simulink model "RobotDelta_NMPC"  (R2025b)
settings: Solver=daessc  StartTime=0.0  StopTime=10  MaxStep=1e-2  RelTol=1e-3
PreLoadFcn:
  | if isempty(which('RobotDelta_Params')), run(fullfile(fileparts(get_param(bdroot,'FileName')),'..','tools','rd_addpath.m')); end; RobotDelta_Params;
InitFcn:
  | RobotDelta_Params; addpath(fullfile(rd_root(), 'work'));
undefined symbols (not defined in the file): G, Nmpc, RobotDelta_IK, RobotDelta_Traj, smiData, Traj, X, Y, Z
libraries: sm_lib x256, nesl_utility x13
(part 1 of 6)
settings Model: Creator=nguye  LastModifiedBy=nguye

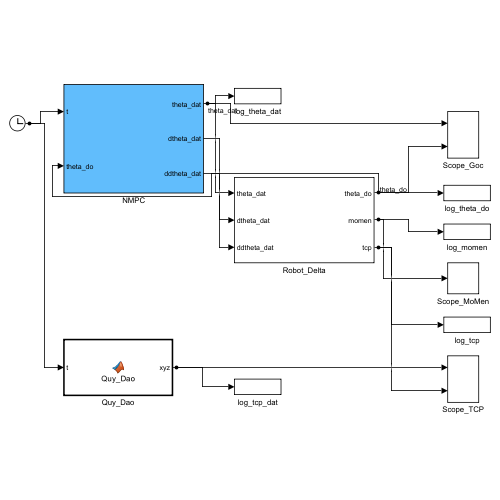
[thumbnail: Simulink's stored preview of the top-level diagram]
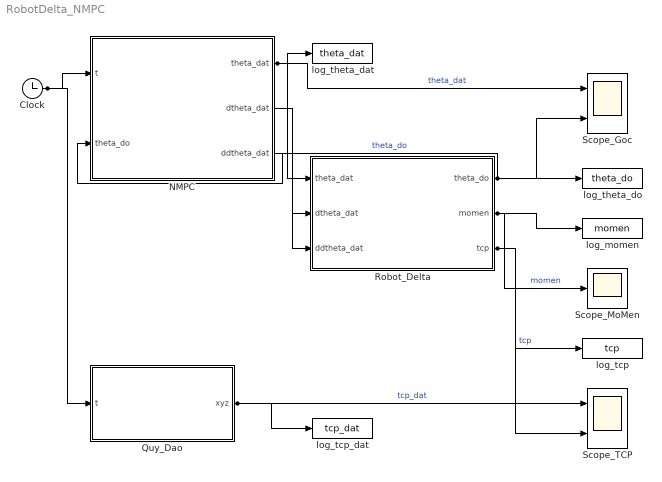
== system RobotDelta_NMPC ==
  Clock : Clock
  NMPC : Subsystem
  Quy_Dao : MATLAB Function  TreatAsAtomicUnit=on
  Robot_Delta : Subsystem
  Scope_Goc : Scope  NumInputPorts=2
  Scope_MoMen : Scope
  Scope_TCP : Scope  NumInputPorts=2
  log_momen : ToWorkspace  VariableName=momen  SaveFormat=Timeseries  SampleTime=-1
  log_tcp : ToWorkspace  VariableName=tcp  SaveFormat=Timeseries  SampleTime=-1
  log_tcp_dat : ToWorkspace  VariableName=tcp_dat  SaveFormat=Timeseries  SampleTime=-1
  log_theta_dat : ToWorkspace  VariableName=theta_dat  SaveFormat=Timeseries  SampleTime=-1
  log_theta_do : ToWorkspace  VariableName=theta_do  SaveFormat=Timeseries  SampleTime=-1
  wires:
  Robot_Delta/2(momen) -> Scope_MoMen/1, log_momen/1  "momen"
  Clock/1 -> Quy_Dao/1(t), NMPC/1(t)
  Quy_Dao/1(xyz) -> Scope_TCP/1, log_tcp_dat/1  "tcp_dat"
  Robot_Delta/1(theta_do) -> Scope_Goc/2, log_theta_do/1, NMPC/2(theta_do)  "theta_do"
  Robot_Delta/3(tcp) -> Scope_TCP/2, log_tcp/1  "tcp"
  NMPC/1(theta_dat) -> Scope_Goc/1, Robot_Delta/1(theta_dat), log_theta_dat/1  "theta_dat"
  NMPC/2(dtheta_dat) -> Robot_Delta/2(dtheta_dat)
  NMPC/3(ddtheta_dat) -> Robot_Delta/3(ddtheta_dat)

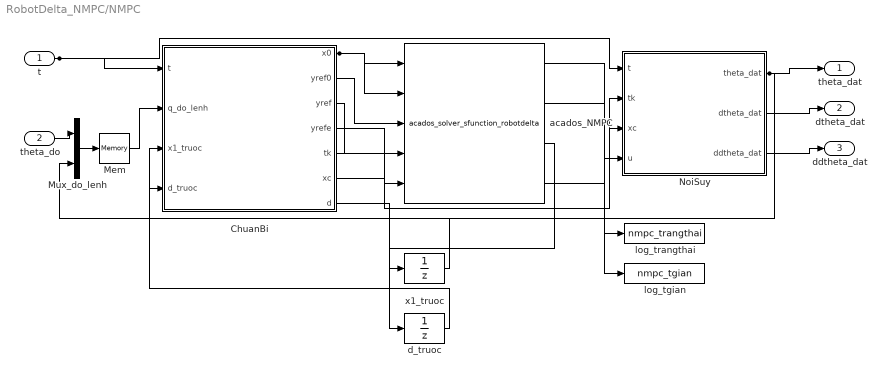
== system RobotDelta_NMPC/NMPC ==
  t : Inport
  theta_do : Inport  Port=2
  ChuanBi : MATLAB Function  TreatAsAtomicUnit=on
  Mem : Memory  InitialCondition=repmat(RobotDelta_IK(RobotDelta_Traj(0, Traj), G), 2, 1)
  Mux_do_lenh : Mux  Inputs=2
  NoiSuy : MATLAB Function  TreatAsAtomicUnit=on
  acados_NMPC : S-Function  FunctionName=acados_solver_sfunction_robotdelta  SFunctionDeploymentMode=off  EnableBusSupport=off
  d_truoc : UnitDelay  InitialCondition=zeros(3,1)  SampleTime=Nmpc.Ts  HasFrameUpgradeWarning=on
  log_tgian : ToWorkspace  VariableName=nmpc_tgian  SaveFormat=Timeseries  SampleTime=-1
  log_trangthai : ToWorkspace  VariableName=nmpc_trangthai  SaveFormat=Timeseries  SampleTime=-1
  x1_truoc : UnitDelay  InitialCondition=[RobotDelta_IK(RobotDelta_Traj(0, Traj), G)*pi/180; 0; 0; 0]  SampleTime=Nmpc.Ts  HasFrameUpgradeWarning=on
  theta_dat : Outport
  dtheta_dat : Outport  Port=2
  ddtheta_dat : Outport  Port=3
  wires:
  t/1 -> ChuanBi/1(t), NoiSuy/1(t)
  theta_do/1 -> Mux_do_lenh/1
  NoiSuy/1(theta_dat) -> Mux_do_lenh/2, theta_dat/1
  Mux_do_lenh/1 -> Mem/1
  Mem/1 -> ChuanBi/2(q_do_lenh)
  x1_truoc/1 -> ChuanBi/3(x1_truoc)
  d_truoc/1 -> ChuanBi/4(d_truoc)
  ChuanBi/7(d) -> d_truoc/1
  ChuanBi/1(x0) -> acados_NMPC/1, acados_NMPC/2
  ChuanBi/2(yref0) -> acados_NMPC/3
  ChuanBi/3(yref) -> acados_NMPC/4
  ChuanBi/4(yrefe) -> acados_NMPC/5
  acados_NMPC/3 -> x1_truoc/1
  ChuanBi/5(tk) -> NoiSuy/2(tk)
  ChuanBi/6(xc) -> NoiSuy/3(xc)
  acados_NMPC/1 -> NoiSuy/4(u)
  acados_NMPC/2 -> log_trangthai/1
  acados_NMPC/4 -> log_tgian/1
  NoiSuy/2(dtheta_dat) -> dtheta_dat/1
  NoiSuy/3(ddtheta_dat) -> ddtheta_dat/1

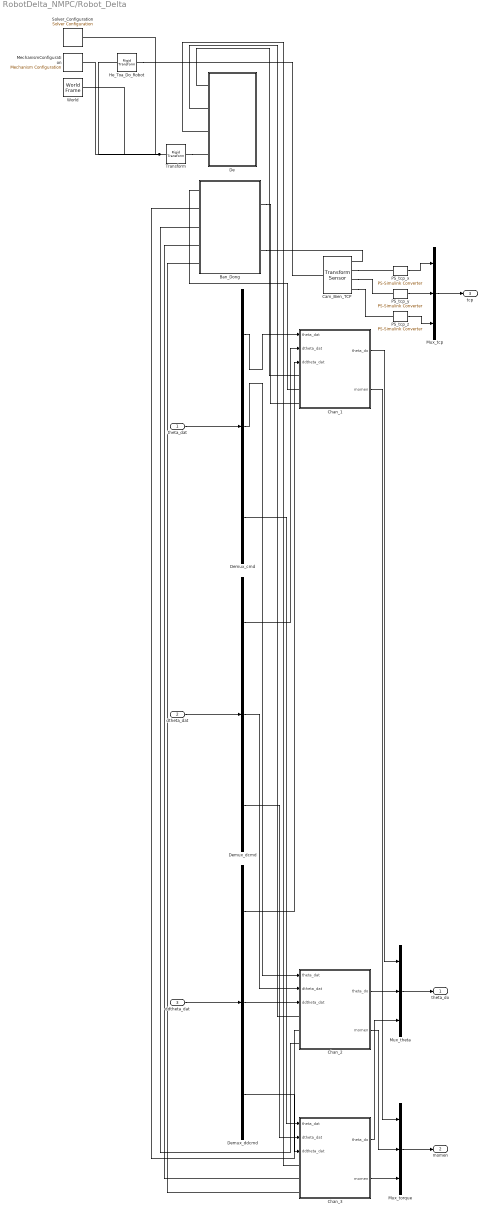
== system RobotDelta_NMPC/Robot_Delta ==
  theta_dat : Inport
  dtheta_dat : Inport  Port=2
  ddtheta_dat : Inport  Port=3
  Ban_Dong : Subsystem
  Cam_Bien_TCP : sm_lib/Frames and Transforms/Transform Sensor  MeasurementFrame=World  RotationSequence=XYX  SenseAngle=off  SenseAxis=off  SenseQ=off  SenseR=off  SenseRotationSequence=off  SenseOmegaX=off  SenseOmegaY=off  SenseOmegaZ=off  SenseOmega=off  SenseQDot=off  SenseRDot=off  SenseRotationSequenceDot=off  SenseAlphaX=off  SenseAlphaY=off  SenseAlphaZ=off  SenseAlpha=off  SenseQDDot=off  SenseRDDot=off  SenseX=on  SenseY=on  SenseZ=on  SenseXYZ=off  SenseRad=off  SenseAzim=off  SenseDist=off  SenseInc=off  SenseXDot=off  SenseYDot=off  SenseZDot=off  SenseXYZDot=off  SenseRadDot=off  SenseAzimDot=off  SenseDistDot=off  SenseIncDot=off  SenseXDDot=off  SenseYDDot=off  SenseZDDot=off  SenseXYZDDot=off  SenseRadDDot=off  SenseAzimDDot=off  SenseDistDDot=off  SenseIncDDot=off
  Chan_1 : Subsystem
  Chan_2 : Subsystem
  Chan_3 : Subsystem
  De : Subsystem
  Demux_cmd : Demux  Outputs=3
  Demux_dcmd : Demux  Outputs=3
  Demux_ddcmd : Demux  Outputs=3
  He_Toa_Do_Robot : sm_lib/Frames and Transforms/Rigid Transform  RotationMethod=None  FollAlignAxisA=+X  BaseAlignAxisA=+Y  FollAlignAxisB=+Y  BaseAlignAxisB=+Z  RotationStandardAxis=+Z  RotationAngle=0  RotationAngleUnits=deg  RotationArbitraryAxis=[0 0 1]  RotationSequenceAxes=FollowerAxes  RotationSequence=XYX  RotationSequenceAngles=[0 0 0]  RotationSequenceAnglesUnits=deg  RotationMatrix=[1 0 0;0 1 0;0 0 1]  Quaternion=[1 0 0 0]  TranslationMethod=Cartesian  TranslationCartesianOffset=G.origin  TranslationCartesianOffsetUnits=m  TranslationStandardAxis=+Z  TranslationStandardOffset=0  TranslationStandardOffsetUnits=m  TranslationROffset=0  TranslationROffsetUnits=m  TranslationThetaOffset=0  TranslationThetaOffsetUnits=deg  TranslationZOffset=0  TranslationZOffsetUnits=m
  MechanismConfiguration : sm_lib/Utilities/Mechanism Configuration  UniformGravity=Constant  GravityVector=[0 0 -9.80665]  GravityVectorUnits=m/s^2  LinearizationDelta=0.001  JointModeTransitionNonlinearIterations=2
  Mux_tcp : Mux  Inputs=3
  Mux_theta : Mux  Inputs=3
  Mux_torque : Mux  Inputs=3
  PS_tcp_x : nesl_utility/PS-Simulink Converter  PhysicalDomain=network_engine_domain  SubClassName=ps_output  LeftPortType=input  RightPortType=output  PseudoPeriodic=off  Frequencies=[]  VectorFormat=inherit  Unit=m  AffineConversion=off
  PS_tcp_y : nesl_utility/PS-Simulink Converter  PhysicalDomain=network_engine_domain  SubClassName=ps_output  LeftPortType=input  RightPortType=output  PseudoPeriodic=off  Frequencies=[]  VectorFormat=inherit  Unit=m  AffineConversion=off
  PS_tcp_z : nesl_utility/PS-Simulink Converter  PhysicalDomain=network_engine_domain  SubClassName=ps_output  LeftPortType=input  RightPortType=output  PseudoPeriodic=off  Frequencies=[]  VectorFormat=inherit  Unit=m  AffineConversion=off
  Solver_Configuration : nesl_utility/Solver Configuration  PhysicalDomain=network_engine_domain  SubClassName=solver  LeftPortType=input  RightPortType=generic  Tones=[]  Harmonics=[]  SimulateNoise=off  Profile=off  UseLocalSampling=off  EnableSwitchedLinearOptims=on  FrequencyDomain=off  UseCCode=off  RelTol=0.001  AbsTol=0.001  MinStep=1e-09  ToWorkspace=off  RevertToSquareIcSolve=off  NumHomotopyIterations=100  PhasorMode=off  PhasorModeNumHarmonics=1  ConsistencySolver=NEWTON_XTOL_AFTER_FTOL  IndexReductionMethod=DerivativeReplacement  DoDC=off  ResidualTolerance=1e-09  ConsistencyTolSource=GLOBAL  ConsistencyAbsTol=0.001  ConsistencyRelTol=0.001  ConsistencyTolFactor=0.001  UseLocalSolver=off  LocalSolverChoice=NE_BACKWARD_EULER_ADVANCER  ResolveIndetEquations=on  FunctionEvalNumThread=1  LocalSolverSampleTime=0.001  DoFixedCost=off  MaxNonlinIter=3  MaxModeIter=2  ComputeImpulses=off  ImpulseIterations=2  LinearAlgebra=auto  LinearAlgebraNumThread=0  EquationFormulation=NE_TIME_EF  DelaysMemoryBudget=1024  AutomaticFiltering=on  FilteringTimeConstant=0.001  PartitionStorageMethod=AS_NEEDED  PartitionMemoryBudget=1024  PartitionMethod=ROBUST  MultibodyUseLocalSolver=off  MultibodyLocalSolverChoice=ODE1  MultibodyLocalSolverSampleTime=0.001
  Transform : sm_lib/Frames and Transforms/Rigid Transform  RotationMethod=ArbitraryAxis  FollAlignAxisA=+X  BaseAlignAxisA=+Y  FollAlignAxisB=+Y  BaseAlignAxisB=+Z  RotationStandardAxis=+Z  RotationAngle=smiData.RigidTransform(126).angle  RotationAngleUnits=rad  RotationArbitraryAxis=smiData.RigidTransform(126).axis  RotationSequenceAxes=FollowerAxes  RotationSequence=XYX  RotationSequenceAngles=[0 0 0]  RotationSequenceAnglesUnits=deg  RotationMatrix=[1 0 0;0 1 0;0 0 1]  Quaternion=[1 0 0 0]  TranslationMethod=Cartesian  TranslationCartesianOffset=smiData.RigidTransform(126).translation  TranslationCartesianOffsetUnits=mm  TranslationStandardAxis=+Z  TranslationStandardOffset=0  TranslationStandardOffsetUnits=m  TranslationROffset=0  TranslationROffsetUnits=m  TranslationThetaOffset=0  TranslationThetaOffsetUnits=deg  TranslationZOffset=0  TranslationZOffsetUnits=m
  World : sm_lib/Frames and Transforms/World Frame
  theta_do : Outport
  momen : Outport  Port=2
  tcp : Outport  Port=3
  wires:
  ddtheta_dat/1 -> Demux_ddcmd/1
  Demux_cmd/2 -> Chan_2/1(theta_dat)
  theta_dat/1 -> Demux_cmd/1
  Mux_torque/1 -> momen/1
  dtheta_dat/1 -> Demux_dcmd/1
  Demux_dcmd/1 -> Chan_1/2(dtheta_dat)
  Chan_1/2(momen) -> Mux_torque/1
  Demux_cmd/1 -> Chan_1/1(theta_dat)
  Demux_dcmd/2 -> Chan_2/2(dtheta_dat)
  Chan_2/2(momen) -> Mux_torque/2
  Mux_theta/1 -> theta_do/1
  Demux_cmd/3 -> Chan_3/1(theta_dat)
  Demux_dcmd/3 -> Chan_3/2(dtheta_dat)
  Demux_ddcmd/1 -> Chan_1/3(ddtheta_dat)
  Chan_1/1(theta_do) -> Mux_theta/1
  Demux_ddcmd/2 -> Chan_2/3(ddtheta_dat)
  PS_tcp_y/1 -> Mux_tcp/2
  Demux_ddcmd/3 -> Chan_3/3(ddtheta_dat)
  Chan_2/1(theta_do) -> Mux_theta/2
  Chan_3/1(theta_do) -> Mux_theta/3
  Chan_3/2(momen) -> Mux_torque/3
  PS_tcp_z/1 -> Mux_tcp/3
  PS_tcp_x/1 -> Mux_tcp/1
  Mux_tcp/1 -> tcp/1
  connections:
  He_Toa_Do_Robot/LConn1 -- Solver_Configuration/RConn1 -- MechanismConfiguration/RConn1 -- Transform/LConn1 -- World/RConn1
  De/LConn3 -- Chan_3/LConn1
  Cam_Bien_TCP/RConn3 -- PS_tcp_y/LConn1
  Ban_Dong/LConn5 -- Chan_3/LConn3
  He_Toa_Do_Robot/RConn1 -- Cam_Bien_TCP/LConn1
  Transform/RConn1 -- De/LConn4
  De/LConn2 -- Chan_2/LConn1
  De/LConn1 -- Chan_1/LConn1
  Ban_Dong/LConn4 -- Chan_3/LConn2
  Ban_Dong/LConn3 -- Chan_2/LConn3
  Ban_Dong/LConn2 -- Chan_2/LConn2
  Ban_Dong/LConn1 -- Chan_1/LConn2
  Ban_Dong/RConn1 -- Chan_1/LConn3
  Ban_Dong/RConn2 -- Cam_Bien_TCP/RConn1
  Cam_Bien_TCP/RConn2 -- PS_tcp_x/LConn1
  Cam_Bien_TCP/RConn4 -- PS_tcp_z/LConn1

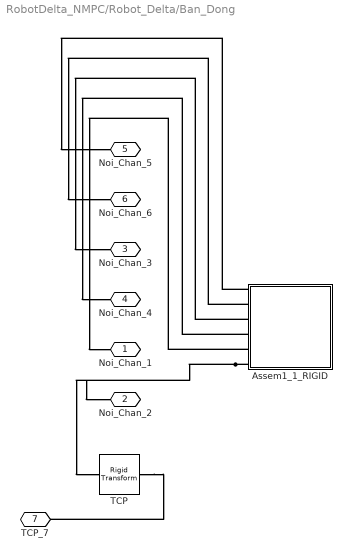
== system RobotDelta_NMPC/Robot_Delta/Ban_Dong ==
  Assem1_1_RIGID : Subsystem
  TCP : sm_lib/Frames and Transforms/Rigid Transform  RotationMethod=RotationMatrix  FollAlignAxisA=+X  BaseAlignAxisA=+Y  FollAlignAxisB=+Y  BaseAlignAxisB=+Z  RotationStandardAxis=+Z  RotationAngle=0  RotationAngleUnits=deg  RotationArbitraryAxis=[0 0 1]  RotationSequenceAxes=FollowerAxes  RotationSequence=XYX  RotationSequenceAngles=[0 0 0]  RotationSequenceAnglesUnits=deg  RotationMatrix=G.tcpRot  Quaternion=[1 0 0 0]  TranslationMethod=Cartesian  TranslationCartesianOffset=G.tcpLocal  TranslationCartesianOffsetUnits=m  TranslationStandardAxis=+Z  TranslationStandardOffset=0  TranslationStandardOffsetUnits=m  TranslationROffset=0  TranslationROffsetUnits=m  TranslationThetaOffset=0  TranslationThetaOffsetUnits=deg  TranslationZOffset=0  TranslationZOffsetUnits=m
  Noi_Chan_1 : PMIOPort  Side=Left
  Noi_Chan_2 : PMIOPort  Port=2  Side=Right
  Noi_Chan_3 : PMIOPort  Port=3  Side=Left
  Noi_Chan_4 : PMIOPort  Port=4  Side=Left
  Noi_Chan_5 : PMIOPort  Port=5  Side=Left
  Noi_Chan_6 : PMIOPort  Port=6  Side=Left
  TCP_7 : PMIOPort  Port=7  Side=Right
  connections:
  TCP/RConn1 -- TCP_7/RConn1
  Assem1_1_RIGID/LConn2 -- Noi_Chan_6/RConn1
  Assem1_1_RIGID/LConn6 -- TCP/LConn1 -- Noi_Chan_2/RConn1
  Assem1_1_RIGID/LConn5 -- Noi_Chan_1/RConn1
  Assem1_1_RIGID/LConn3 -- Noi_Chan_3/RConn1
  Assem1_1_RIGID/LConn4 -- Noi_Chan_4/RConn1
  Assem1_1_RIGID/LConn1 -- Noi_Chan_5/RConn1

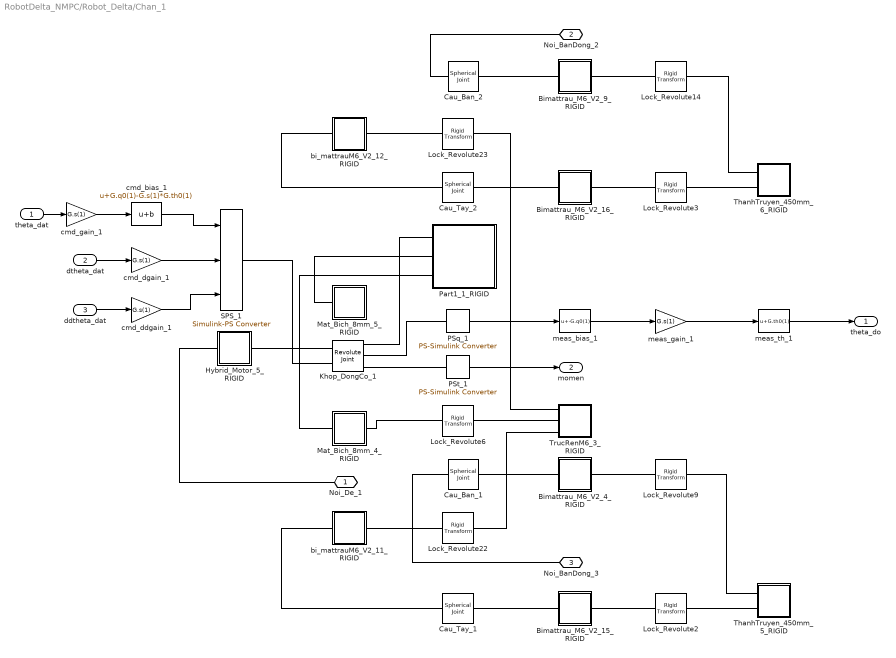
== system RobotDelta_NMPC/Robot_Delta/Chan_1 ==
  theta_dat : Inport
  dtheta_dat : Inport  Port=2
  ddtheta_dat : Inport  Port=3
  Bimattrau_M6_V2_15_RIGID : Subsystem
  Bimattrau_M6_V2_16_RIGID : Subsystem
  Bimattrau_M6_V2_4_RIGID : Subsystem
  Bimattrau_M6_V2_9_RIGID : Subsystem
  Cau_Ban_1 : sm_lib/Joints/Spherical Joint  JointMode=Normal  CompositeWrenchDir=FollowerOnBase  CompositeWrenchFrame=BaseFrame  SenseConstraintForce=off  SenseConstraintTorque=off  SenseTotalForce=off  SenseTotalTorque=off  PositionTargetSpecify=off  PositionTargetPriority=High  PositionTargetRotationMethod=None  PositionTargetFollAlignAxisA=+X  PositionTargetBaseAlignAxisA=+Y  PositionTargetFollAlignAxisB=+Y  PositionTargetBaseAlignAxisB=+Z  PositionTargetRotationStandardAxis=+Z  PositionTargetRotationAngle=0  PositionTargetRotationAngleUnits=deg  PositionTargetRotationArbitraryAxis=[0 0 1]  PositionTargetRotationSequenceAxes=FollowerAxes  PositionTargetRotationSequence=XYX  PositionTargetRotationSequenceAngles=[0 0 0]  PositionTargetRotationSequenceAnglesUnits=deg  PositionTargetRotationMatrix=[1 0 0;0 1 0;0 0 1]  PositionTargetQuaternion=[1 0 0 0]  VelocityTargetSpecify=off  VelocityTargetPriority=High  VelocityTargetValue=[0 0 0]  VelocityTargetValueUnits=deg/s  VelocityTargetInFollowerFrame=on  EqPosRotationMethod=None  EqPosFollAlignAxisA=+X  EqPosBaseAlignAxisA=+Y  EqPosFollAlignAxisB=+Y  EqPosBaseAlignAxisB=+Z  EqPosRotationStandardAxis=+Z  EqPosRotationAngle=0  EqPosRotationAngleUnits=deg  EqPosRotationArbitraryAxis=[0 0 1]  EqPosRotationSequenceAxes=FollowerAxes  EqPosRotationSequence=XYX  EqPosRotationSequenceAngles=[0 0 0]  EqPosRotationSequenceAnglesUnits=deg  EqPosRotationMatrix=[1 0 0;0 1 0;0 0 1]  EqPosQuaternion=[1 0 0 0]  SpringStiffness=0  SpringStiffnessUnits=N*m/deg  DampingCoefficient=0  DampingCoefficientUnits=N*m/(deg/s)  LowerLimitSpecify=off  LowerLimitBound=15  LowerLimitBoundUnits=deg  LowerLimitStiffness=1e4  LowerLimitStiffnessUnits=N*m/deg  LowerLimitDamping=10  LowerLimitDampingUnits=N*m/(deg/s)  LowerLimitTransitionRegionWidth=0.1  LowerLimitTransitionRegionWidthUnits=deg  UpperLimitSpecify=off  UpperLimitBound=45  UpperLimitBoundUnits=deg  UpperLimitStiffness=1e4  UpperLimitStiffnessUnits=N*m/deg  UpperLimitDamping=10  UpperLimitDampingUnits=N*m/(deg/s)  UpperLimitTransitionRegionWidth=0.1  UpperLimitTransitionRegionWidthUnits=deg  TorqueActuationMode=NoTorque  ActuateTorqueX=off  ActuateTorqueY=off  ActuateTorqueZ=off  ActuateTorque=off  ActuationFrame=BaseFrame  SensePosition=off  SenseVelocityX=off  SenseVelocityY=off  SenseVelocityZ=off  SenseVelocity=off  SenseAccelerationX=off  SenseAccelerationY=off  SenseAccelerationZ=off  SenseAcceleration=off  SenseLowerLimitTorqueMag=off  SenseUpperLimitTorqueMag=off  SensingFrame=BaseFrame
  Cau_Ban_2 : sm_lib/Joints/Spherical Joint  JointMode=Normal  CompositeWrenchDir=FollowerOnBase  CompositeWrenchFrame=BaseFrame  SenseConstraintForce=off  SenseConstraintTorque=off  SenseTotalForce=off  SenseTotalTorque=off  PositionTargetSpecify=off  PositionTargetPriority=High  PositionTargetRotationMethod=None  PositionTargetFollAlignAxisA=+X  PositionTargetBaseAlignAxisA=+Y  PositionTargetFollAlignAxisB=+Y  PositionTargetBaseAlignAxisB=+Z  PositionTargetRotationStandardAxis=+Z  PositionTargetRotationAngle=0  PositionTargetRotationAngleUnits=deg  PositionTargetRotationArbitraryAxis=[0 0 1]  PositionTargetRotationSequenceAxes=FollowerAxes  PositionTargetRotationSequence=XYX  PositionTargetRotationSequenceAngles=[0 0 0]  PositionTargetRotationSequenceAnglesUnits=deg  PositionTargetRotationMatrix=[1 0 0;0 1 0;0 0 1]  PositionTargetQuaternion=[1 0 0 0]  VelocityTargetSpecify=off  VelocityTargetPriority=High  VelocityTargetValue=[0 0 0]  VelocityTargetValueUnits=deg/s  VelocityTargetInFollowerFrame=on  EqPosRotationMethod=None  EqPosFollAlignAxisA=+X  EqPosBaseAlignAxisA=+Y  EqPosFollAlignAxisB=+Y  EqPosBaseAlignAxisB=+Z  EqPosRotationStandardAxis=+Z  EqPosRotationAngle=0  EqPosRotationAngleUnits=deg  EqPosRotationArbitraryAxis=[0 0 1]  EqPosRotationSequenceAxes=FollowerAxes  EqPosRotationSequence=XYX  EqPosRotationSequenceAngles=[0 0 0]  EqPosRotationSequenceAnglesUnits=deg  EqPosRotationMatrix=[1 0 0;0 1 0;0 0 1]  EqPosQuaternion=[1 0 0 0]  SpringStiffness=0  SpringStiffnessUnits=N*m/deg  DampingCoefficient=0  DampingCoefficientUnits=N*m/(deg/s)  LowerLimitSpecify=off  LowerLimitBound=15  LowerLimitBoundUnits=deg  LowerLimitStiffness=1e4  LowerLimitStiffnessUnits=N*m/deg  LowerLimitDamping=10  LowerLimitDampingUnits=N*m/(deg/s)  LowerLimitTransitionRegionWidth=0.1  LowerLimitTransitionRegionWidthUnits=deg  UpperLimitSpecify=off  UpperLimitBound=45  UpperLimitBoundUnits=deg  UpperLimitStiffness=1e4  UpperLimitStiffnessUnits=N*m/deg  UpperLimitDamping=10  UpperLimitDampingUnits=N*m/(deg/s)  UpperLimitTransitionRegionWidth=0.1  UpperLimitTransitionRegionWidthUnits=deg  TorqueActuationMode=NoTorque  ActuateTorqueX=off  ActuateTorqueY=off  ActuateTorqueZ=off  ActuateTorque=off  ActuationFrame=BaseFrame  SensePosition=off  SenseVelocityX=off  SenseVelocityY=off  SenseVelocityZ=off  SenseVelocity=off  SenseAccelerationX=off  SenseAccelerationY=off  SenseAccelerationZ=off  SenseAcceleration=off  SenseLowerLimitTorqueMag=off  SenseUpperLimitTorqueMag=off  SensingFrame=BaseFrame
  Cau_Tay_1 : sm_lib/Joints/Spherical Joint  JointMode=Normal  CompositeWrenchDir=FollowerOnBase  CompositeWrenchFrame=BaseFrame  SenseConstraintForce=off  SenseConstraintTorque=off  SenseTotalForce=off  SenseTotalTorque=off  PositionTargetSpecify=off  PositionTargetPriority=High  PositionTargetRotationMethod=None  PositionTargetFollAlignAxisA=+X  PositionTargetBaseAlignAxisA=+Y  PositionTargetFollAlignAxisB=+Y  PositionTargetBaseAlignAxisB=+Z  PositionTargetRotationStandardAxis=+Z  PositionTargetRotationAngle=0  PositionTargetRotationAngleUnits=deg  PositionTargetRotationArbitraryAxis=[0 0 1]  PositionTargetRotationSequenceAxes=FollowerAxes  PositionTargetRotationSequence=XYX  PositionTargetRotationSequenceAngles=[0 0 0]  PositionTargetRotationSequenceAnglesUnits=deg  PositionTargetRotationMatrix=[1 0 0;0 1 0;0 0 1]  PositionTargetQuaternion=[1 0 0 0]  VelocityTargetSpecify=off  VelocityTargetPriority=High  VelocityTargetValue=[0 0 0]  VelocityTargetValueUnits=deg/s  VelocityTargetInFollowerFrame=on  EqPosRotationMethod=None  EqPosFollAlignAxisA=+X  EqPosBaseAlignAxisA=+Y  EqPosFollAlignAxisB=+Y  EqPosBaseAlignAxisB=+Z  EqPosRotationStandardAxis=+Z  EqPosRotationAngle=0  EqPosRotationAngleUnits=deg  EqPosRotationArbitraryAxis=[0 0 1]  EqPosRotationSequenceAxes=FollowerAxes  EqPosRotationSequence=XYX  EqPosRotationSequenceAngles=[0 0 0]  EqPosRotationSequenceAnglesUnits=deg  EqPosRotationMatrix=[1 0 0;0 1 0;0 0 1]  EqPosQuaternion=[1 0 0 0]  SpringStiffness=0  SpringStiffnessUnits=N*m/deg  DampingCoefficient=0  DampingCoefficientUnits=N*m/(deg/s)  LowerLimitSpecify=off  LowerLimitBound=15  LowerLimitBoundUnits=deg  LowerLimitStiffness=1e4  LowerLimitStiffnessUnits=N*m/deg  LowerLimitDamping=10  LowerLimitDampingUnits=N*m/(deg/s)  LowerLimitTransitionRegionWidth=0.1  LowerLimitTransitionRegionWidthUnits=deg  UpperLimitSpecify=off  UpperLimitBound=45  UpperLimitBoundUnits=deg  UpperLimitStiffness=1e4  UpperLimitStiffnessUnits=N*m/deg  UpperLimitDamping=10  UpperLimitDampingUnits=N*m/(deg/s)  UpperLimitTransitionRegionWidth=0.1  UpperLimitTransitionRegionWidthUnits=deg  TorqueActuationMode=NoTorque  ActuateTorqueX=off  ActuateTorqueY=off  ActuateTorqueZ=off  ActuateTorque=off  ActuationFrame=BaseFrame  SensePosition=off  SenseVelocityX=off  SenseVelocityY=off  SenseVelocityZ=off  SenseVelocity=off  SenseAccelerationX=off  SenseAccelerationY=off  SenseAccelerationZ=off  SenseAcceleration=off  SenseLowerLimitTorqueMag=off  SenseUpperLimitTorqueMag=off  SensingFrame=BaseFrame
  Cau_Tay_2 : sm_lib/Joints/Spherical Joint  JointMode=Normal  CompositeWrenchDir=FollowerOnBase  CompositeWrenchFrame=BaseFrame  SenseConstraintForce=off  SenseConstraintTorque=off  SenseTotalForce=off  SenseTotalTorque=off  PositionTargetSpecify=off  PositionTargetPriority=High  PositionTargetRotationMethod=None  PositionTargetFollAlignAxisA=+X  PositionTargetBaseAlignAxisA=+Y  PositionTargetFollAlignAxisB=+Y  PositionTargetBaseAlignAxisB=+Z  PositionTargetRotationStandardAxis=+Z  PositionTargetRotationAngle=0  PositionTargetRotationAngleUnits=deg  PositionTargetRotationArbitraryAxis=[0 0 1]  PositionTargetRotationSequenceAxes=FollowerAxes  PositionTargetRotationSequence=XYX  PositionTargetRotationSequenceAngles=[0 0 0]  PositionTargetRotationSequenceAnglesUnits=deg  PositionTargetRotationMatrix=[1 0 0;0 1 0;0 0 1]  PositionTargetQuaternion=[1 0 0 0]  VelocityTargetSpecify=off  VelocityTargetPriority=High  VelocityTargetValue=[0 0 0]  VelocityTargetValueUnits=deg/s  VelocityTargetInFollowerFrame=on  EqPosRotationMethod=None  EqPosFollAlignAxisA=+X  EqPosBaseAlignAxisA=+Y  EqPosFollAlignAxisB=+Y  EqPosBaseAlignAxisB=+Z  EqPosRotationStandardAxis=+Z  EqPosRotationAngle=0  EqPosRotationAngleUnits=deg  EqPosRotationArbitraryAxis=[0 0 1]  EqPosRotationSequenceAxes=FollowerAxes  EqPosRotationSequence=XYX  EqPosRotationSequenceAngles=[0 0 0]  EqPosRotationSequenceAnglesUnits=deg  EqPosRotationMatrix=[1 0 0;0 1 0;0 0 1]  EqPosQuaternion=[1 0 0 0]  SpringStiffness=0  SpringStiffnessUnits=N*m/deg  DampingCoefficient=0  DampingCoefficientUnits=N*m/(deg/s)  LowerLimitSpecify=off  LowerLimitBound=15  LowerLimitBoundUnits=deg  LowerLimitStiffness=1e4  LowerLimitStiffnessUnits=N*m/deg  LowerLimitDamping=10  LowerLimitDampingUnits=N*m/(deg/s)  LowerLimitTransitionRegionWidth=0.1  LowerLimitTransitionRegionWidthUnits=deg  UpperLimitSpecify=off  UpperLimitBound=45  UpperLimitBoundUnits=deg  UpperLimitStiffness=1e4  UpperLimitStiffnessUnits=N*m/deg  UpperLimitDamping=10  UpperLimitDampingUnits=N*m/(deg/s)  UpperLimitTransitionRegionWidth=0.1  UpperLimitTransitionRegionWidthUnits=deg  TorqueActuationMode=NoTorque  ActuateTorqueX=off  ActuateTorqueY=off  ActuateTorqueZ=off  ActuateTorque=off  ActuationFrame=BaseFrame  SensePosition=off  SenseVelocityX=off  SenseVelocityY=off  SenseVelocityZ=off  SenseVelocity=off  SenseAccelerationX=off  SenseAccelerationY=off  SenseAccelerationZ=off  SenseAcceleration=off  SenseLowerLimitTorqueMag=off  SenseUpperLimitTorqueMag=off  SensingFrame=BaseFrame
  Hybrid_Motor_5_RIGID : Subsystem
  Khop_DongCo_1 : sm_lib/Joints/Revolute Joint  JointMode=Normal  CompositeWrenchDir=FollowerOnBase  CompositeWrenchFrame=BaseFrame  SenseConstraintForce=off  SenseConstraintTorque=off  SenseTotalForce=off  SenseTotalTorque=off  PositionTargetSpecify=on  PositionTargetPriority=Low  PositionTargetValue=smiData.RevoluteJoint(16).Rz.Pos  PositionTargetValueUnits=deg  VelocityTargetSpecify=off  VelocityTargetPriority=High  VelocityTargetValue=0  VelocityTargetValueUnits=deg/s  EquilibriumPosition=0  EquilibriumPositionUnits=deg  SpringStiffness=0  SpringStiffnessUnits=N*m/deg  DampingCoefficient=0  DampingCoefficientUnits=N*m/(deg/s)  LowerLimitSpecify=off  LowerLimitBound=-90  LowerLimitBoundUnits=deg  LowerLimitStiffness=1e4  LowerLimitStiffnessUnits=N*m/deg  LowerLimitDamping=10  LowerLimitDampingUnits=N*m/(deg/s)  LowerLimitTransitionRegionWidth=0.1  LowerLimitTransitionRegionWidthUnits=deg  UpperLimitSpecify=off  UpperLimitBound=90  UpperLimitBoundUnits=deg  UpperLimitStiffness=1e4  UpperLimitStiffnessUnits=N*m/deg  UpperLimitDamping=10  UpperLimitDampingUnits=N*m/(deg/s)  UpperLimitTransitionRegionWidth=0.1  UpperLimitTransitionRegionWidthUnits=deg  TorqueActuationMode=ComputedTorque  MotionActuationMode=InputMotion  SensePosition=on  SenseVelocity=off  SenseAcceleration=off  SenseTorqueForce=on  SenseLowerLimitTorqueForce=off  SenseUpperLimitTorqueForce=off
  Lock_Revolute14 : sm_lib/Frames and Transforms/Rigid Transform  RotationMethod=StandardAxis  FollAlignAxisA=+X  BaseAlignAxisA=+Y  FollAlignAxisB=+Y  BaseAlignAxisB=+Z  RotationStandardAxis=+Z  RotationAngle=-113.31644323681007  RotationAngleUnits=deg  RotationArbitraryAxis=[0 0 1]  RotationSequenceAxes=FollowerAxes  RotationSequence=XYX  RotationSequenceAngles=[0 0 0]  RotationSequenceAnglesUnits=deg  RotationMatrix=[1 0 0;0 1 0;0 0 1]  Quaternion=[1 0 0 0]  TranslationMethod=Cartesian  TranslationCartesianOffset=[0 0 0]  TranslationCartesianOffsetUnits=m  TranslationStandardAxis=+Z  TranslationStandardOffset=0  TranslationStandardOffsetUnits=m  TranslationROffset=0  TranslationROffsetUnits=m  TranslationThetaOffset=0  TranslationThetaOffsetUnits=deg  TranslationZOffset=0  TranslationZOffsetUnits=m
  Lock_Revolute2 : sm_lib/Frames and Transforms/Rigid Transform  RotationMethod=StandardAxis  FollAlignAxisA=+X  BaseAlignAxisA=+Y  FollAlignAxisB=+Y  BaseAlignAxisB=+Z  RotationStandardAxis=+Z  RotationAngle=14.860535928527009  RotationAngleUnits=deg  RotationArbitraryAxis=[0 0 1]  RotationSequenceAxes=FollowerAxes  RotationSequence=XYX  RotationSequenceAngles=[0 0 0]  RotationSequenceAnglesUnits=deg  RotationMatrix=[1 0 0;0 1 0;0 0 1]  Quaternion=[1 0 0 0]  TranslationMethod=Cartesian  TranslationCartesianOffset=[0 0 0]  TranslationCartesianOffsetUnits=m  TranslationStandardAxis=+Z  TranslationStandardOffset=0  TranslationStandardOffsetUnits=m  TranslationROffset=0  TranslationROffsetUnits=m  TranslationThetaOffset=0  TranslationThetaOffsetUnits=deg  TranslationZOffset=0  TranslationZOffsetUnits=m
  Lock_Revolute22 : sm_lib/Frames and Transforms/Rigid Transform  RotationMethod=StandardAxis  FollAlignAxisA=+X  BaseAlignAxisA=+Y  FollAlignAxisB=+Y  BaseAlignAxisB=+Z  RotationStandardAxis=+Z  RotationAngle=-2.2853446130210751  RotationAngleUnits=deg  RotationArbitraryAxis=[0 0 1]  RotationSequenceAxes=FollowerAxes  RotationSequence=XYX  RotationSequenceAngles=[0 0 0]  RotationSequenceAnglesUnits=deg  RotationMatrix=[1 0 0;0 1 0;0 0 1]  Quaternion=[1 0 0 0]  TranslationMethod=Cartesian  TranslationCartesianOffset=[0 0 -0.00099999999999987512]  TranslationCartesianOffsetUnits=m  TranslationStandardAxis=+Z  TranslationStandardOffset=0  TranslationStandardOffsetUnits=m  TranslationROffset=0  TranslationROffsetUnits=m  TranslationThetaOffset=0  TranslationThetaOffsetUnits=deg  TranslationZOffset=0  TranslationZOffsetUnits=m
  Lock_Revolute23 : sm_lib/Frames and Transforms/Rigid Transform  RotationMethod=StandardAxis  FollAlignAxisA=+X  BaseAlignAxisA=+Y  FollAlignAxisB=+Y  BaseAlignAxisB=+Z  RotationStandardAxis=+Z  RotationAngle=-92.994645805531547  RotationAngleUnits=deg  RotationArbitraryAxis=[0 0 1]  RotationSequenceAxes=FollowerAxes  RotationSequence=XYX  RotationSequenceAngles=[0 0 0]  RotationSequenceAnglesUnits=deg  RotationMatrix=[1 0 0;0 1 0;0 0 1]  Quaternion=[1 0 0 0]  TranslationMethod=Cartesian  TranslationCartesianOffset=[0 0 -0.00099999999999991675]  TranslationCartesianOffsetUnits=m  TranslationStandardAxis=+Z  TranslationStandardOffset=0  TranslationStandardOffsetUnits=m  TranslationROffset=0  TranslationROffsetUnits=m  TranslationThetaOffset=0  TranslationThetaOffsetUnits=deg  TranslationZOffset=0  TranslationZOffsetUnits=m
  Lock_Revolute3 : sm_lib/Frames and Transforms/Rigid Transform  RotationMethod=StandardAxis  FollAlignAxisA=+X  BaseAlignAxisA=+Y  FollAlignAxisB=+Y  BaseAlignAxisB=+Z  RotationStandardAxis=+Z  RotationAngle=139.1416458636977  RotationAngleUnits=deg  RotationArbitraryAxis=[0 0 1]  RotationSequenceAxes=FollowerAxes  RotationSequence=XYX  RotationSequenceAngles=[0 0 0]  RotationSequenceAnglesUnits=deg  RotationMatrix=[1 0 0;0 1 0;0 0 1]  Quaternion=[1 0 0 0]  TranslationMethod=Cartesian  TranslationCartesianOffset=[0 0 0]  TranslationCartesianOffsetUnits=m  TranslationStandardAxis=+Z  TranslationStandardOffset=0  TranslationStandardOffsetUnits=m  TranslationROffset=0  TranslationROffsetUnits=m  TranslationThetaOffset=0  TranslationThetaOffsetUnits=deg  TranslationZOffset=0  TranslationZOffsetUnits=m
  Lock_Revolute6 : sm_lib/Frames and Transforms/Rigid Transform  RotationMethod=StandardAxis  FollAlignAxisA=+X  BaseAlignAxisA=+Y  FollAlignAxisB=+Y  BaseAlignAxisB=+Z  RotationStandardAxis=+Z  RotationAngle=12.352912697906175  RotationAngleUnits=deg  RotationArbitraryAxis=[0 0 1]  RotationSequenceAxes=FollowerAxes  RotationSequence=XYX  RotationSequenceAngles=[0 0 0]  RotationSequenceAnglesUnits=deg  RotationMatrix=[1 0 0;0 1 0;0 0 1]  Quaternion=[1 0 0 0]  TranslationMethod=Cartesian  TranslationCartesianOffset=[0 0 0]  TranslationCartesianOffsetUnits=m  TranslationStandardAxis=+Z  TranslationStandardOffset=0  TranslationStandardOffsetUnits=m  TranslationROffset=0  TranslationROffsetUnits=m  TranslationThetaOffset=0  TranslationThetaOffsetUnits=deg  TranslationZOffset=0  TranslationZOffsetUnits=m
  Lock_Revolute9 : sm_lib/Frames and Transforms/Rigid Transform  RotationMethod=StandardAxis  FollAlignAxisA=+X  BaseAlignAxisA=+Y  FollAlignAxisB=+Y  BaseAlignAxisB=+Z  RotationStandardAxis=+Z  RotationAngle=163.92313017276496  RotationAngleUnits=deg  RotationArbitraryAxis=[0 0 1]  RotationSequenceAxes=FollowerAxes  RotationSequence=XYX  RotationSequenceAngles=[0 0 0]  RotationSequenceAnglesUnits=deg  RotationMatrix=[1 0 0;0 1 0;0 0 1]  Quaternion=[1 0 0 0]  TranslationMethod=Cartesian  TranslationCartesianOffset=[0 0 0]  TranslationCartesianOffsetUnits=m  TranslationStandardAxis=+Z  TranslationStandardOffset=0  TranslationStandardOffsetUnits=m  TranslationROffset=0  TranslationROffsetUnits=m  TranslationThetaOffset=0  TranslationThetaOffsetUnits=deg  TranslationZOffset=0  TranslationZOffsetUnits=m
  Mat_Bich_8mm_4_RIGID : Subsystem
  Mat_Bich_8mm_5_RIGID : Subsystem
  PSq_1 : nesl_utility/PS-Simulink Converter  PhysicalDomain=network_engine_domain  SubClassName=ps_output  LeftPortType=input  RightPortType=output  PseudoPeriodic=off  Frequencies=[]  VectorFormat=inherit  Unit=deg  AffineConversion=off
  PSt_1 : nesl_utility/PS-Simulink Converter  PhysicalDomain=network_engine_domain  SubClassName=ps_output  LeftPortType=input  RightPortType=output  PseudoPeriodic=off  Frequencies=[]  VectorFormat=inherit  Unit=N*m  AffineConversion=off
  Part1_1_RIGID : Subsystem
  SPS_1 : nesl_utility/Simulink-PS Converter  PhysicalDomain=network_engine_domain  SubClassName=ps_input  LeftPortType=input  RightPortType=output  PseudoPeriodic=off  Frequencies=[]  NoiseDistribution=none  NoiseParameters=[]  Unit=deg  AffineConversion=off  FilteringAndDerivatives=provide  SimscapeFilterOrder=1  InputFilterTimeConstant=0.001  UdotUserProvided=2
  ThanhTruyen_450mm_5_RIGID : Subsystem
  ThanhTruyen_450mm_6_RIGID : Subsystem
  TrucRenM6_3_RIGID : Subsystem
  bi_mattrauM6_V2_11_RIGID : Subsystem
  bi_mattrauM6_V2_12_RIGID : Subsystem
  cmd_bias_1 : Bias  Bias=G.q0(1)-G.s(1)*G.th0(1)  SaturateOnIntegerOverflow=off
  cmd_ddgain_1 : Gain  Gain=G.s(1)
  cmd_dgain_1 : Gain  Gain=G.s(1)
  cmd_gain_1 : Gain  Gain=G.s(1)
  meas_bias_1 : Bias  Bias=-G.q0(1)  SaturateOnIntegerOverflow=off
  meas_gain_1 : Gain  Gain=G.s(1)
  meas_th_1 : Bias  Bias=G.th0(1)  SaturateOnIntegerOverflow=off
  Noi_De_1 : PMIOPort  Side=Left
  Noi_BanDong_2 : PMIOPort  Port=2  Side=Left
  Noi_BanDong_3 : PMIOPort  Port=3  Side=Left
  theta_do : Outport
  momen : Outport  Port=2
  wires:
  PSt_1/1 -> momen/1
  cmd_ddgain_1/1 -> SPS_1/3
  cmd_bias_1/1 -> SPS_1/1
  cmd_gain_1/1 -> cmd_bias_1/1
  theta_dat/1 -> cmd_gain_1/1
  dtheta_dat/1 -> cmd_dgain_1/1
  cmd_dgain_1/1 -> SPS_1/2
  ddtheta_dat/1 -> cmd_ddgain_1/1
  PSq_1/1 -> meas_bias_1/1
  meas_th_1/1 -> theta_do/1
  meas_bias_1/1 -> meas_gain_1/1
  meas_gain_1/1 -> meas_th_1/1
  connections:
  Noi_BanDong_2/RConn1 -- Cau_Ban_2/LConn1
  SPS_1/RConn1 -- Khop_DongCo_1/LConn2
  Hybrid_Motor_5_RIGID/RConn1 -- Khop_DongCo_1/LConn1
  bi_mattrauM6_V2_12_RIGID/LConn1 -- Cau_Tay_2/LConn1
  Mat_Bich_8mm_5_RIGID/LConn1 -- Part1_1_RIGID/LConn2
  Mat_Bich_8mm_4_RIGID/LConn1 -- Part1_1_RIGID/LConn3
  Noi_De_1/RConn1 -- Hybrid_Motor_5_RIGID/LConn1
  bi_mattrauM6_V2_12_RIGID/RConn1 -- Lock_Revolute23/LConn1
  bi_mattrauM6_V2_11_RIGID/LConn1 -- Cau_Tay_1/LConn1
  Khop_DongCo_1/RConn1 -- Part1_1_RIGID/LConn1
  Khop_DongCo_1/RConn2 -- PSq_1/LConn1
  Khop_DongCo_1/RConn3 -- PSt_1/LConn1
  Bimattrau_M6_V2_9_RIGID/RConn1 -- Lock_Revolute14/LConn1
  Mat_Bich_8mm_4_RIGID/RConn1 -- Lock_Revolute6/LConn1
  Lock_Revolute2/RConn1 -- ThanhTruyen_450mm_5_RIGID/LConn2
  bi_mattrauM6_V2_11_RIGID/RConn1 -- Lock_Revolute22/LConn1
  Cau_Ban_2/RConn1 -- Bimattrau_M6_V2_9_RIGID/LConn1
  Lock_Revolute23/RConn1 -- TrucRenM6_3_RIGID/LConn1
  Cau_Tay_2/RConn1 -- Bimattrau_M6_V2_16_RIGID/LConn1
  Lock_Revolute6/RConn1 -- TrucRenM6_3_RIGID/LConn2
  Cau_Ban_1/RConn1 -- Bimattrau_M6_V2_4_RIGID/LConn1
  Lock_Revolute22/RConn1 -- TrucRenM6_3_RIGID/LConn3
  Cau_Tay_1/RConn1 -- Bimattrau_M6_V2_15_RIGID/LConn1
  Noi_BanDong_3/RConn1 -- Cau_Ban_1/LConn1
  Bimattrau_M6_V2_16_RIGID/RConn1 -- Lock_Revolute3/LConn1
  Bimattrau_M6_V2_4_RIGID/RConn1 -- Lock_Revolute9/LConn1
  Bimattrau_M6_V2_15_RIGID/RConn1 -- Lock_Revolute2/LConn1
  Lock_Revolute14/RConn1 -- ThanhTruyen_450mm_6_RIGID/LConn1
  Lock_Revolute3/RConn1 -- ThanhTruyen_450mm_6_RIGID/LConn2
  Lock_Revolute9/RConn1 -- ThanhTruyen_450mm_5_RIGID/LConn1
